simulink model "bidirection_buck_boost"  (R2025a)
settings: Solver=VariableStepAuto  StartTime=0.0  StopTime=0.05  MaxStep=1e-7  RelTol=1e-3
libraries: ee_lib x36, nesl_utility x29, fl_lib x26, spsPWMGeneratorDCDCLib x8, spsMeanLib x2, batteryecm_lib x1
settings Model: Creator=GNKRISHNAN  LastModifiedBy=GNKRISHNAN

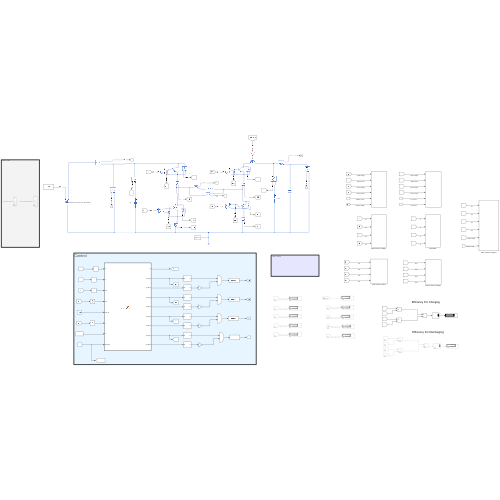
[thumbnail: Simulink's stored preview of the top-level diagram]
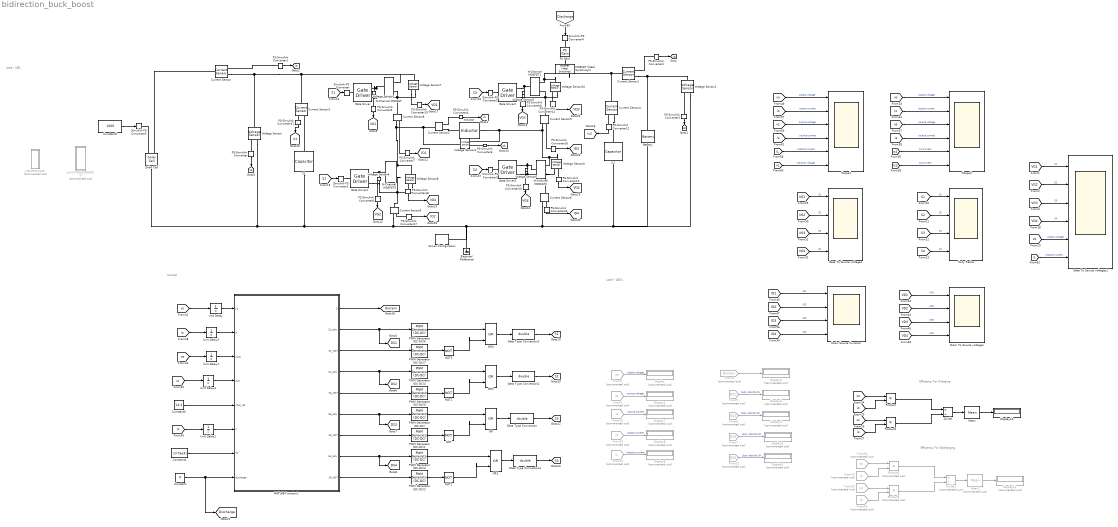
== system bidirection_buck_boost ==
  note: Load - LED
  note: Load - LED's
  note: Control
  note: Efficiency For Charging
  note: Efficiency For Discharging
  Battery : batteryecm_lib/Battery  Vnom=12 V  prm_dir=simscape.enum.battery.prm_dir.disabled  R1_dis=2 Ohm  R1_ch=2 Ohm  R1=4.9e-3 Ohm  prm_AH=simscape.enum.battery.prm_AH.infinite  AH=7.2 A*hr  V1=11.5 V  AH1=25 A*hr  prm_R2=simscape.enum.battery.prm_R2.disabled  R2=2000 Ohm  Tmeas=298.15 K  charge_measurement_port=simscape.enum.battery.enable.no  prm_dyn=simscape.enum.battery.prm_dyn.off  Rp1=0.005 Ohm  tau1=30 s  Rp2=0.005 Ohm  tau2=30 s  Rp3=0.005 Ohm  tau3=30 s  Rp4=0.005 Ohm  tau4=30 s  Rp5=0.005 Ohm  tau5=30 s  prm_fade=simscape.enum.battery.prm_fade.disabled  N_fade=100  AH_fade=45 A*hr  R1_fade=2.02 Ohm  R1_ch_fade=2.02 Ohm  V1_fade=10.35 V  prm_age=simscape.enum.battery.prm_age.disabled  prm_age_OCV=simscape.enum.battery.prm_age_OCV.OCV  OCV_age=0.9  SOC_age=60  Tmeas_age=298.15 K  delta_time_age_vec=[0] d  temperature_age_vec=[273] K  OCV_scaling_age=2.2134e6  OCV_offset_age=1.632e6  temp_exp_age=0.515833569 V  t_exp_age=0.75  Vnom_T2=12 V  R1_T2=2.2 Ohm  R1_T2_dis=2.2 Ohm  R1_T2_ch=2.2 Ohm  V1_T2=11.4 V  R2_T2=2200 Ohm  Rp1_T2=0.005 Ohm  tau1_T2=30 s  Rp2_T2=0.005 Ohm  tau2_T2=30 s  Rp3_T2=0.005 Ohm  tau3_T2=30 s  Rp4_T2=0.005 Ohm  tau4_T2=30 s  Rp5_T2=0.005 Ohm  tau5_T2=30 s  Tmeas2=273.15 K  thermal_port=simscape.enum.thermaleffects.omit  thermal_mass=30000 J/K  i_specify=off  i_priority=None  i=0 A  i_nominal_specify=off  i_nominal_value=1  i_nominal_unit=A  v_specify=off  v_priority=None  v=0 V  v_nominal_specify=off  v_nominal_value=1  v_nominal_unit=V  charge_specify=off  charge_priority=High  charge=50 A*hr  charge_nominal_specify=off  charge_nominal_value=1  charge_nominal_unit=A*hr  num_cycles_specify=off  num_cycles_priority=High  num_cycles=0  num_cycles_nominal_specify=off  num_cycles_nominal_value=1  num_cycles_nominal_unit=1  temperature_specify=off  temperature_priority=High  temperature=298.15 K  temperature_nominal_specify=off  temperature_nominal_value=1  temperature_nominal_unit=K
      settings: LibrarySourceBlock=batt_lib/Cells/Battery
  C1 : fl_lib/Electrical/Electrical Elements/Capacitor  c=100e-6 F  r=1e-6 Ohm  g=0 1/Ohm  i_specify=off  i_priority=High  i=1 A  i_nominal_specify=off  i_nominal_value=1  i_nominal_unit=A  v_specify=off  v_priority=Low  v=50 V  v_nominal_specify=off  v_nominal_value=1  v_nominal_unit=V  vc_specify=off  vc_priority=High  vc=50 V  vc_nominal_specify=off  vc_nominal_value=1  vc_nominal_unit=V
  C2 : fl_lib/Electrical/Electrical Elements/Capacitor  c=488e-6 F  r=1e-6 Ohm  g=0 1/Ohm  i_specify=off  i_priority=High  i=1 A  i_nominal_specify=off  i_nominal_value=1  i_nominal_unit=A  v_specify=off  v_priority=Low  v=12 V  v_nominal_specify=off  v_nominal_value=1  v_nominal_unit=V  vc_specify=off  vc_priority=High  vc=12 V  vc_nominal_specify=off  vc_nominal_value=1  vc_nominal_unit=V
  Constant : Constant  Value=0
  Constant4 : Constant  Value=1/(75e3)
  Constant5 : Constant  Value=1000
  Constant6 : Constant  Value=14.2
  Current Sensor{,1..6,8..9} (9 alike) : fl_lib/Electrical/Electrical Sensors/Current Sensor
  Data Type Conversion{,1..3} (4 alike) : DataTypeConversion  OutDataTypeStr=double  SaturateOnIntegerOverflow=off  RndMeth=Floor
  Display{,1..9,11} (11 alike) : Display  Commented=on
      Display11 settings: Format=bank
  Display10 : Display
      settings: Format=bank
  Divide : Product  Inputs=*/
  Divide1 : Product  Commented=on  Inputs=*/
  Drain Source Currents : Scope  NumInputPorts=4
      settings: ActiveDisplayString=4  ActiveDisplayYMinimum=-1.5306429258777277  ActiveDisplayYMaximum=0.21907576990254851  DataLoggingVariableName=ScopeData5
  Drain To Source voltages : Scope  NumInputPorts=4
      settings: ActiveDisplayYMinimum=-4.5564425884228816  ActiveDisplayYMaximum=38.582414890367822  DataLoggingVariableName=ScopeData4
  Duty Ratios : Scope  NumInputPorts=4
      settings: ActiveDisplayYMinimum=0.9  ActiveDisplayYMaximum=1.1
  Electrical Reference : fl_lib/Electrical/Electrical Elements/Electrical Reference
  From19 : From  Commented=on  GotoTag=is  TagVisibility=global
  From20 : From  Commented=on  GotoTag=io  TagVisibility=global
  From21 : From  Commented=on  GotoTag=iL  TagVisibility=global
  From22 : From  Commented=on  GotoTag=DS4  TagVisibility=global
  From4 : From  Commented=on  GotoTag=vo  TagVisibility=global
  From5 : From  Commented=on  GotoTag=vs  TagVisibility=global
  From51 : From  Commented=on  GotoTag=vs  TagVisibility=global
  From52 : From  Commented=on  GotoTag=is  TagVisibility=global
  From53 : From  Commented=on  GotoTag=vo  TagVisibility=global
  From54 : From  Commented=on  GotoTag=io  TagVisibility=global
  From6 : From  Commented=on  GotoTag=DS2  TagVisibility=global
  From7 : From  Commented=on  GotoTag=DS3  TagVisibility=global
  From8 : From  Commented=on  GotoTag=Dintern  TagVisibility=global
  From9 : From  Commented=on  GotoTag=DS1  TagVisibility=global
  Gate Driver{,1..3} (4 alike) : ee_lib/Semiconductors & Converters/Gate Driver  port_option=ee.enum.controlport.ps  uHigh=2.0 V  uLow=0.8 V  uHighValue=0.7  uLowValue=0.3  vHigh=15 V  vLow=0 V  tHigh=500 ns  tLow=0 ns  parameterization=ee.enum.semiconductors.gateDriverParam.outputImpedance  rHigh=2 Ohm  rLow=2 Ohm  tRise=20 ns  tFall=20 ns  cLoad=10 nF  ZonTime_specify=off  ZonTime_priority=None  ZonTime=0 s  ZoffTime_specify=off  ZoffTime_priority=None  ZoffTime=0 s
      settings: InternalSimscapePortConfiguration="{\"Bottom\":[],\"Left\":[{\"id\":\"u\",\"label\":\"u\",\"type\":\"input\"}],\"Right\":[{\"id\":\"G\",\"label\":\"G\",\"type\":\"foundation.electrical.electrical\"},{\"id\":\"S\",\"label\":\"S\",\"type\":\"foundation.electrical.electrical\"}],\"Top\":[]}"
  Gate To Source voltages : Scope  NumInputPorts=4
      settings: ActiveDisplayString=4  ActiveDisplayYMinimum=-2.1171010981224692  ActiveDisplayYMaximum=16.901953933343137  DataLoggingVariableName=ScopeData2
  Gate To Source voltages1 : Scope  NumInputPorts=6
      settings: ActiveDisplayString=6  ActiveDisplayYMinimum=-4.895588317884668  ActiveDisplayYMaximum=-0.48622530824491572
  Inductor : ee_lib/Passive/Inductor  l=150e-6 H  enable_L_tol=ee.enum.toleranceApplication.none  L_tol=20  tol_distribution=ee.enum.toleranceDistribution.uniform  nSigma=4  r=0 Ohm  g=1e-9 1/Ohm  enable_operating_limits=ee.enum.enable.no  operating_limit_action=ee.enum.passive.reportOpLim.warn  max_working_current=1 A  power_rating=1 W  i_L_specify=off  i_L_priority=High  i_L=2.5 A  i_L_nominal_specify=on  i_L_nominal_value=3  i_L_nominal_unit=A
  L1HZ-5780100000000 : Subsystem  Commented=on
  LXK2PW14V00 : Subsystem  Commented=on
      settings: PortSchema="{\"entries\":[{\"content\":{\"sides\":[{\"content\":{},\"type\":\"ConnectorPlacement.EquallySpacedRectSide\",\"uuid\":\"20fc5c96-5131-4911-af40-90c1653f2349\"},{\"content\":{\"side\":\"RIGHT\"},\"type\":\"ConnectorPlacement.EquallySpacedRectSide\",\"uuid\":\"84d94f68-b5bd-4d52-87d0-e2c404d7394b\"},{\"content\":{\"connectorIds\":[\"LConn1\"],\"side\":\"TOP\"},\"type\":\"ConnectorPlacement.EquallySpacedRectSide\",\"uuid\":\"fbb55fab-e1b4-4776-8e6f-d36497a875a9\"},{\"content\":{\"connectorIds\":[\"RConn1\"],\"side\":\"BOTTOM\"},\"type\":\"ConnectorPlacement.EquallySpacedRectSide\",\"uuid\":\"0f47366a-6e94-42f9-9b64-329c1064e3d3\"}]},\"type\":\"ConnectorPlacement.EquallySpacedConnector\",\"uuid\":\"9fc36618-202f-478c-8e37-58b0074959b4\"}],\"packageUris\":[\"http://schema.mathworks.com/mf0/Connector/R2020b\"],\"version\":\"1.0\"}"
  MATLAB Function1 : MATLAB Function  TreatAsAtomicUnit=on  SystemSampleTime=1/(75e3)
  "MOSFET (Ideal, Switching)4" : ee_lib/Semiconductors & Converters/MOSFET (Ideal, Switching)  port_option=ee.enum.controlport.ps  Rds=0.01 Ohm  Goff=1e-6 1/Ohm  Vth=0.5 V  diode_param=ee.enum.semiconductors.protectionDiode.nodynamics  diode_Vf=0.8 V  diode_Ron=0.001 Ohm  diode_Goff=1e-5 1/Ohm  diode_C=50e-9 F  diode_iRM=-235 A  diode_iF=300 A  diode_idot=-50 A/us  diode_trr_param=ee.enum.converters.diodeReverseParam.trr_factor  diode_trr_factor=3  diode_trr=15 us  diode_Qrr=1500 s*uA  ids_specify=off  ids_priority=None  ids=0 A  ids_nominal_specify=off  ids_nominal_value=1  ids_nominal_unit=A  vds_specify=off  vds_priority=None  vds=0 V  vds_nominal_specify=off  vds_nominal_value=1  vds_nominal_unit=V  vgs_specify=off  vgs_priority=None  vgs=0 V  vgs_nominal_specify=off  vgs_nominal_value=1  vgs_nominal_unit=V  thermal_loss_option=ee.enum.converters.thermalLossOption.constantvalues  Von_data=[0, 1.8, 3.2, 6, 10, 16; 0, 2, 5.5, 9.5, 15, 25] V  Tj=[298.15, 448.15] K  Iout_data=[0, 20, 40, 60, 80, 100] A  Eon_data=[0, 55.04, 124.57, 235.53, 362.12; 0, 71.25, 161.25, 304.88, 468.75] * 1e-6 J  Eoff_data=[0, 18, 30, 56.1, 76.5; 0, 22.5, 37.5, 70.13, 95.63] * 1e-6 J  Eon_data_3D=[zeros(2, 5, 3)] J  Eoff_data_3D=[zeros(2, 5, 3)] J  Tj_loss=[298.15, 448.15] K  Iout_data_loss=[0, 10, 20, 30, 40] A  tabulateWithVds=false  Vds_loss=[0, 150, 300] V  Eon_scalar=22.86e-3 J  Eoff_scalar=17.14e-3 J  Voff=300 V  Iout_scalar=600 A  useCurrentFromPreviousCycle=false  useVoltageFromPreviousCycle=false  diodeModelType=ee.enum.converters.diodeModelType.pwl  diodeTableType=ee.enum.diode.tableType.IfMat  diode_ReverseIVType=ee.enum.diode.diodeReverseIV.constant  diode_IfMat=[.07, .12, .19, 1.75, 4.24, 7.32, 11.2; .16, .3, .72, 2.14, 4.02, 6.35, 9.12] A  diode_VfMat=[.9, 1.15, 1.25, 1.5, 1.75, 2.17, 2.6, 2.85; .58, .68, .75, 1.1, 1.38, 1.77, 2.27, 2.7] V  diode_TjVec=[25, 125] degC  diode_VfVec=[.5, .7, .9, 1.3, 1.7, 2.1, 2.5] V  diode_IfVec=[.1, .2, .5, 1, 2, 4, 7, 10] A  diode_IrMat=[1e-06, 2e-06, 5e-06, 1e-05, 2.5e-05, 5e-05, .0001; 2e-06, 5e-06, 1e-05, 4e-05, 8e-05, .0002, .0005] A  diode_VrMat=[10, 100, 200, 250, 300, 325, 350; 10, 70, 160, 220, 270, 300, 320] V  diode_VrVec=[10, 20, 40, 50, 70, 80, 100] V  diode_IrVec=[1e-06, 2e-06, 5e-06, 1e-05, 2e-05, 5e-05, .0001] A  diode_Vr=-600 V  diode_Ls=150 nH  diode_Erec=0.03 J  diode_rec_loss_model=ee.enum.diode.reverseRecoveryModel.fixed  diode_ErecVal=0 J  diode_scaleWithIandV=true  diode_ErecMat=zeros(2, 3) J  diode_TjrecVec=[298.15, 398.15] K  diode_IfrecVec=[.1, 1, 10] A  diode_IrecVal=10 A  diode_VrecVal=10 V  diode_tFilter=1 / 1000 / 100 s  separateThermalPortForDiode=false  thermal_network_parameterization=ee.enum.thermalNetworkTopology.external  Rth=[.03, .2] K/W  Rth_Cauer=[.03, .1, .2] K/W  Rth_Foster=[.08, .14, .22, .16] K/W  thermal_mass_parameterization=ee.enum.thermalNetwork.timeconstant  thermal_mass=[3, 25] J/K  thermal_mass_Cauer=[3, 10, 25] J/K  thermal_mass_Foster=[.001, .005, .05, .5] J/K  thermal_time_constant=[.1, 5] s  thermal_time_constant_Cauer=[.1, 1, 5] s  thermal_time_constant_Foster=[7e-05, .0007, .01, .08] s  thermal_mass_initial_temperatures=[25, 25] degC  thermal_mass_initial_temperatures_Cauer=[25, 25, 25] degC  junction_thermal_mass=0.1 J/K  Tvec_initial_Foster=[25, 25, 25, 25] degC  RthDiode=[.03, .2] K/W  RthCauerDiode=[.03, .1, .2] K/W  RthFosterDiode=[.03, .2] K/W  thermalMassDiode=[3, 25] J/K  thermalMassCauerDiode=[3, 10, 25] J/K  thermalMassFosterDiode=[33, 50] J/K  thermalTauDiode=[.1, 5] s  thermalTauCauerDiode=[.1, 1, 5] s  thermalTauFosterDiode=[1, 10] s  thermalMassInitTempDiode=[25, 25] degC  thermalMassInitTempCauerDiode=[25, 25, 25] degC  junctionthermalMassDiode=0.1 J/K  TVecInitialFosterDiode=[25, 25, 25, 25] degC  no_thermal_network=0  mosfet_junction_temperature_specify=off  mosfet_junction_temperature_priority=None  mosfet_junction_temperature=25 degC  mosfet_junction_temperature_nominal_specify=off  mosfet_junction_temperature_nominal_value=1  mosfet_junction_temperature_nominal_unit=degC  diode_junction_temperature_specify=off  diode_junction_temperature_priority=None  diode_junction_temperature=25 degC  diode_junction_temperature_nominal_specify=off  diode_junction_temperature_nominal_value=1  diode_junction_temperature_nominal_unit=degC  Qj_specify=off  Qj_priority=None  Qj=0 W  Qj_nominal_specify=off  Qj_nominal_value=1  Qj_nominal_unit=W  accumulatedSwitchingLosses_specify=off  accumulatedSwitchingLosses_priority=None  accumulatedSwitchingLosses=0 J
  Mean : spsMeanLib/Mean  Freq=100e3  Vinit=0.5  Ts=0
  Mean1 : spsMeanLib/Mean  Commented=on  Freq=100e3  Vinit=0.5  Ts=0
  N-Channel MOSFET{,1..3} (4 alike) : ee_lib/Semiconductors & Converters/N-Channel MOSFET  paramTerminal=ee.enum.mosfet.numberOfTerminals.three  parameterization=ee.enum.mosfet.parameterization.datasheet  Beta=5.0 A/V^2  Rds=17.5 mOhm  Id=49.0 A  Vgs=20 V  Vth=4.0 V  Vth0=1.7 V  lam=0 1/V  gamma_vth=0.5 V^(1/2)  phib=0.5 V  Vth1=1.9071 V  Vbs1=-1 V  Vth2=2.066 V  Vbs2=-2 V  Tmeas=25 degC  Vgs_vec=[-1, -.5, 2, 3, 4, 5] V  Vds_vec=[0, 2, 4, 8, 12, 16, 20] V  Vbs_vec=[0, -4, -6, -12] V  T_vec=[25, 125] degC  Vth_vec=[.4, 1.2, 1.4, 1.45] V  Vth_mat=[.4, .35; 1.2, 1.15; 1.4, 1.35; 1.45, 1.4] V  Ids_mat=[0, 0, 0, 0, 0, 0, 0; 0, 0, 0, 0, 0, 0, 0; 0, .003, .0038, .0043, .0046, .0048, .0049; 0, .0055, .008, .009, .0095, .01, .0101; 0, .0115, .016, .018, .019, .0195, .02; 0, .0152, .0225, .0265, .028, .0295, .03] A  Ids_mat0=[0, 0, 0, 0, 0, 0, 0; 0, 0, 0, 0, 0, 0, 0; 0, .003, .0038, .0043, .0046, .0048, .0049; 0, .0055, .008, .009, .0095, .01, .0101; 0, .0115, .016, .018, .019, .0195, .02; 0, .0152, .0225, .0265, .028, .0295, .03] A  Ids_mat_3D=zeros(6, 7, 2) A  Ids_mat_3D0=zeros(6, 7, 2) A  IV_table_symmetry=ee.enum.mosfet.symmetricNIV.no  RS=0.0001 Ohm  RD=0.01 Ohm  RB=0.001 Ohm  LeadRs=0 Ohm  LeadRd=0 Ohm  LeadRg=0 Ohm  LeadRb=0 Ohm  LS=0 nH  LD=0 nH  LG=0 nH  LB=0 nH  C_param=ee.enum.mosfet.capacitanceParam.fixedciss  C_GS=270 pF  C_GD=80 pF  C_GB=0 pF  C_DS=0 pF  C_iss=1470 pF  C_rss=88 pF  C_oss=360 pF  C_iss_vec=[720, 700, 590, 470, 390, 310] pF  C_rss_vec=[450, 400, 300, 190, 95, 55] pF  C_oss_vec=[900, 810, 690, 420, 270, 170] pF  C_GS_vec=[270, 300, 290, 280, 295, 255] pF  C_GD_vec=[450, 400, 300, 190, 95, 55] pF  C_GB_vec=[270, 300, 290, 280, 295, 255] pF  C_Vgs_vec=0 V  C_DS_vec=[450, 410, 390, 230, 175, 115] pF  C_Vds_vec=[.1, .3, 1, 3, 10, 30] V  V_GS_for_cap_data=0 V  charge_linearity_param=ee.enum.mosfet.cgdLinearity.constant  C_OX=200 pF  V_C_OX=-0.5 V  charge_linearity_param_vgb=ee.enum.mosfet.cgbLinearity.instantly  charge_linearity_param_with_vgb=ee.enum.mosfet.cgbLinearityWithSeparateCgb.instantly  Di_param=ee.enum.mosfet.diodeParam.no  IsDiode=1e-12 A  Vbi=0.6 V  n=1  Cj0Diode=0 pF  TT=50e-9 s  Tmeas_dio=25 degC  TableTypeNoT=ee.enum.mosfet.tableType.IfMat  TableType=ee.enum.diode.tableType.IfMat  IfVec=[.07, .12, .19, 1.75, 4.24, 7.32, 11.2] A  IfMat=[.07, .12, .19, 1.75, 4.24, 7.32, 11.2; .16, .3, .72, 2.14, 4.02, 6.35, 9.12] A  VfVecV=[.9, 1.15, 1.25, 1.5, 1.75, 2.17, 2.6, 2.85] V  VfMatV=[.9, 1.15, 1.25, 1.5, 1.75, 2.17, 2.6, 2.85; .58, .68, .75, 1.1, 1.38, 1.77, 2.27, 2.7] V  TjVec=[25, 125] degC  VfVec=[.5, .7, .9, 1.3, 1.7, 2.1, 2.5] V  IfVecV=[.1, .2, .5, 1, 2, 4, 7, 10] A  diode_Goff=1e-12 1/Ohm  prmDatasheet=ee.enum.temperatureParameterization.none  prmEquCoeff=ee.enum.temperatureParameterization.none  dVth_dT=-6 mV/K  dVth0_dT=-6 mV/K  Rds_T2=0.037 Ohm  BEXDatasheet=-1.5  BEXEquCoeff=-1.5  etaisDatasheet=3  etaisEquCoeff=3  Tmeas2=125 degC  etaisTabulated=3  TdeviceDatasheet=25 degC  TdeviceEquCoeff=25 degC  TdeviceTabulated=25 degC  i_g_specify=off  i_g_priority=None  i_g=0 A  i_g_nominal_specify=off  i_g_nominal_value=1  i_g_nominal_unit=A  i_d_specify=off  i_d_priority=None  i_d=0 A  i_d_nominal_specify=off  i_d_nominal_value=1  i_d_nominal_unit=A  i_b_specify=off  i_b_priority=None  i_b=0 A  i_b_nominal_specify=off  i_b_nominal_value=1  i_b_nominal_unit=A  voltage_gs_specify=off  voltage_gs_priority=None  voltage_gs=0 V  voltage_gs_nominal_specify=off  voltage_gs_nominal_value=1  voltage_gs_nominal_unit=V  voltage_ds_specify=off  voltage_ds_priority=None  voltage_ds=0 V  voltage_ds_nominal_specify=off  voltage_ds_nominal_value=1  voltage_ds_nominal_unit=V  voltage_bs_specify=off  voltage_bs_priority=None  voltage_bs=0 V  voltage_bs_nominal_specify=off  voltage_bs_nominal_value=1  voltage_bs_nominal_unit=V  v_Cgs_specify=off  v_Cgs_priority=High  v_Cgs=0 V  v_Cgs_nominal_specify=off  v_Cgs_nominal_value=1  v_Cgs_nominal_unit=V  v_Cds_specify=off  v_Cds_priority=High  v_Cds=0 V  v_Cds_nominal_specify=off  v_Cds_nominal_value=1  v_Cds_nominal_unit=V  v_Cbs_specify=off  v_Cbs_priority=High  v_Cbs=0 V  v_Cbs_nominal_specify=off  v_Cbs_nominal_value=1  v_Cbs_nominal_unit=V  thermal_network_parameterization=ee.enum.thermalNetworkTopology.junctionCase  Rth=[0, 10] K/W  Rth_Cauer=[1, 3, 10] K/W  Rth_Foster=[.08, .14, .22, .16] K/W  thermal_mass_parameterization=ee.enum.thermalNetwork.timeconstant  thermal_mass=[0, 1] J/K  thermal_mass_Cauer=[.1, .3, 1] J/K  thermal_mass_Foster=[.001, .005, .05, .5] J/K  thermal_time_constant=[0, 10] s  thermal_time_constant_Cauer=[1, 3, 10] s  thermal_time_constant_Foster=[7e-05, .0007, .01, .08] s  thermal_mass_initial_temperatures=[25, 25] degC  thermal_mass_initial_temperatures_Cauer=[25, 25, 25] degC  Tvec_initial_Foster=[25, 25, 25, 25] degC  betaref=18 A/V^2  Vfbref=-1.1 V  gamma=3.5 V^(1/2)  phib2ref=1 V  thesatref=0.4 1/V  alpha=0  Vp=5e-2 V  thesrref=0 1/V  m=8  Tref=25 degC  Rsref=2e-3 Ohm  Rdref=0.17 Ohm  Rgref=8.4 Ohm  Rbref=2e-3 Ohm  Cox=1500 pF  Cgso=100 pF  Cgdo=14 pF  Isref=5.2e-13 A  Cj0=480 pF  Tprm=1  etabet=1.3  Stvfb=5e-4 V/K  Stphib=-8.5e-4 V/K  etasat=1.04  etasr=0.65  etar=0.95  etais=3  Tsim=25 degC  Ig_specify=off  Ig_priority=None  Ig=0 A  Ig_nominal_specify=off  Ig_nominal_value=1  Ig_nominal_unit=nA  Ids_specify=off  Ids_priority=None  Ids=0 A  Ids_nominal_specify=off  Ids_nominal_value=1  Ids_nominal_unit=A  Ib_specify=off  Ib_priority=None  Ib=0 A  Ib_nominal_specify=off  Ib_nominal_value=1  Ib_nominal_unit=uA  V_gs_specify=off  V_gs_priority=None  V_gs=0 V  V_gs_nominal_specify=off  V_gs_nominal_value=1  V_gs_nominal_unit=V  V_ds_specify=off  V_ds_priority=None  V_ds=0 V  V_ds_nominal_specify=off  V_ds_nominal_value=1  V_ds_nominal_unit=V  V_bs_specify=off  V_bs_priority=None  V_bs=0 V  V_bs_nominal_specify=off  V_bs_nominal_value=1  V_bs_nominal_unit=V  QGoverCox_specify=off  QGoverCox_priority=None  QGoverCox=0 V  QGoverCox_nominal_specify=off  QGoverCox_nominal_value=1  QGoverCox_nominal_unit=V  QDoverCox_specify=off  QDoverCox_priority=None  QDoverCox=0 V  QDoverCox_nominal_specify=off  QDoverCox_nominal_value=1  QDoverCox_nominal_unit=V  QBoverCox_specify=off  QBoverCox_priority=None  QBoverCox=0 V  QBoverCox_nominal_specify=off  QBoverCox_nominal_value=1  QBoverCox_nominal_unit=V  T0=[25, 25] degC  T0_Cauer=[25, 25, 25] degC
  NOT{,1..3} (4 alike) : Logic  Operator=NOT  IconShape=distinctive  AllPortsSameDT=off  OutDataTypeStr=boolean
  OR{,1..3} (4 alike) : Logic  Operator=OR  IconShape=distinctive  AllPortsSameDT=off  OutDataTypeStr=boolean
  PS Gain : fl_lib/Physical Signals/Functions/PS Gain  gain=10 V
  PS-Simulink Converter{,1..12,14..20} (20 alike) : nesl_utility/PS-Simulink Converter  PhysicalDomain=network_engine_domain  SubClassName=ps_output  LeftPortType=input  RightPortType=output  PseudoPeriodic=off  Frequencies=[]  VectorFormat=inherit  Unit=inherit  AffineConversion=off
  PWM Generator (DC-DC){,1..7} (8 alike) : spsPWMGeneratorDCDCLib/PWM Generator (DC-DC)  Fsw=75e3  Ts=0
  Product : Product
  Product1 : Product
  Product2 : Product  Commented=on
  Product3 : Product  Commented=on
  Scope1 : Scope  NumInputPorts=6
      settings: ActiveDisplayString=5  ActiveDisplayYMinimum=-17.405950682168605  ActiveDisplayYMaximum=156.65355621450624  DataLoggingVariableName=ScopeData6
  Scope3 : Scope  NumInputPorts=6
      settings: ActiveDisplayYMinimum=-1.5694108173115382  ActiveDisplayYMaximum=14.126143121517581  DataLoggingVariableName=ScopeData3
  Simulink-PS Converter{,1..5} (6 alike) : nesl_utility/Simulink-PS Converter  PhysicalDomain=network_engine_domain  SubClassName=ps_input  LeftPortType=input  RightPortType=output  PseudoPeriodic=off  Frequencies=[]  NoiseDistribution=none  NoiseParameters=[]  Unit=1  AffineConversion=off  FilteringAndDerivatives=provide  SimscapeFilterOrder=1  InputFilterTimeConstant=0.001  UdotUserProvided=0
  Solar Cell : ee_lib/Sources/Solar Cell  PartSpecification="{\"CollectionId\":\"SimscapeElectrical\",\"CollectionVersion\":\"1.0.0\",\"DatasetId\":\"Mitsubishi_Electric|PV_MLU250HC|simscape.electrical.solarCell\",\"DisplayName\":\"Mitsubishi_Electric:PV_MLU250HC\"}"  prm=3  Isc=4.395 % Datasheet derived A  Voc=0.62698 % Datasheet derived V  Is=3.90785352555275e-07 % Datasheet derived A  Is2=2.03851654351426e-09 % Datasheet derived A  Iph=4.39501564800196 % Datasheet derived A  Ir0=1000 % Datasheet derived W/m^2  ec=1.50308795420873 % Datasheet derived  N2=1.46170678478288 % Datasheet derived  Rs=0.00316744030774209 % Datasheet derived Ohm  Rp=887.270164200596 % Datasheet derived Ohm  N_series=60 % Datasheet derived  N_parallel=2 % Datasheet derived  TIPH1=0.000560046095116037 % Datasheet derived 1/K  EG=1.12 % Datasheet derived eV  TXIS1=6.0075926142096 % Datasheet derived  TXIS2=15.9012627985887 % Datasheet derived  TRS1=0.216297310987677 % Datasheet derived  TRP1=0 % Parameter not set  Tmeas=25 % Datasheet derived degC  TFIXED=25 % Datasheet derived degC  thermal_mass=100 % Parameter not set J/K  initial_temperature=25 degC
      settings: AttributesFormatString=Mitsubishi_Electric:PV_MLU250HC
  Solver Configuration : nesl_utility/Solver Configuration  PhysicalDomain=network_engine_domain  SubClassName=solver  LeftPortType=input  RightPortType=generic  Tones=[]  Harmonics=[]  SimulateNoise=off  Profile=off  UseLocalSampling=off  EnableSwitchedLinearOptims=on  FrequencyDomain=off  UseCCode=off  RelTol=0.001  AbsTol=0.001  MinStep=1e-09  ToWorkspace=off  RevertToSquareIcSolve=off  NumHomotopyIterations=100  PhasorMode=off  PhasorModeNumHarmonics=1  ConsistencySolver=NEWTON_XTOL_AFTER_FTOL  IndexReductionMethod=DerivativeReplacement  DoDC=off  ResidualTolerance=1e-09  ConsistencyTolSource=GLOBAL  ConsistencyAbsTol=0.001  ConsistencyRelTol=0.001  ConsistencyTolFactor=0.001  UseLocalSolver=off  LocalSolverChoice=NE_BACKWARD_EULER_ADVANCER  ResolveIndetEquations=on  FunctionEvalNumThread=1  LocalSolverSampleTime=0.001  DoFixedCost=off  MaxNonlinIter=3  MaxModeIter=2  ComputeImpulses=off  ImpulseIterations=2  LinearAlgebra=auto  LinearAlgebraNumThread=0  EquationFormulation=NE_TIME_EF  DelaysMemoryBudget=1024  AutomaticFiltering=on  FilteringTimeConstant=0.001  PartitionStorageMethod=AS_NEEDED  PartitionMemoryBudget=1024  PartitionMethod=ROBUST  MultibodyUseLocalSolver=off  MultibodyLocalSolverChoice=ODE1  MultibodyLocalSolverSampleTime=0.001
  Unit Delay{,1..4} (5 alike) : UnitDelay  SampleTime=-1  HasFrameUpgradeWarning=on
  Voltage Sensor{,1..10} (11 alike) : fl_lib/Electrical/Electrical Sensors/Voltage Sensor
  tag scope: DS1=global, DS2=global, DS3=global, DS4=global, Dintern=global, Discharge=global, ID1=global, ID2=global, ID3=global, ID4=global, S1=global, S2=global, S3=global, S4=global, VD1=global, VD2=global, VD3=global, VD4=global, VG1=global, VG2=global, VG3=global, VG4=global, iL=global, ic1=global, ic2=global, io=global, is=global, vL=global, vo=global, vs=global
  wires:
  From6/1 -> Display4/1  "Duty ratio for S2"
  From22/1 -> Display6/1  "Duty ratio for S4"
  [S2] -> Duty Ratios/2  "S2"
  Unit Delay/1 -> MATLAB Function1/1(Vs)
  From8/1 -> Display2/1
  MATLAB Function1/8(S4_duty) -> PWM Generator (DC-DC)3/1, [DS4]
  Unit Delay1/1 -> MATLAB Function1/3(Vout)
  [vo] -> Unit Delay1/1
  [S1] -> Simulink-PS Converter/1
  [S4] -> Duty Ratios/4  "S4"
  [S3] -> Simulink-PS Converter2/1
  Constant4/1 -> MATLAB Function1/7(Ts)
  PS-Simulink Converter2/1 -> [vo]
  PS-Simulink Converter1/1 -> [is]
  [vs] -> Unit Delay/1
  [S1] -> Duty Ratios/1  "S1"
  Unit Delay2/1 -> MATLAB Function1/6(Il)
  PS-Simulink Converter4/1 -> [iL]
  [S3] -> Duty Ratios/3  "S3"
  From9/1 -> Display3/1  "Duty ratio for S1"
  [iL] -> Unit Delay2/1
  From4/1 -> Display/1  "output voltage"
  MATLAB Function1/6(S3_duty) -> PWM Generator (DC-DC)/1, [DS3]
  [S4] -> Simulink-PS Converter3/1
  PS-Simulink Converter/1 -> [vs]
  PS-Simulink Converter3/1 -> [io]
  From7/1 -> Display5/1  "Duty ratio for S3"
  From5/1 -> Display1/1  "source voltage"
  [S2] -> Simulink-PS Converter1/1
  From20/1 -> Display8/1  "output current"
  From19/1 -> Display7/1  "source current"
  From21/1 -> Display9/1  "inductor current"
  PS-Simulink Converter5/1 -> [VG1]
  PS-Simulink Converter6/1 -> [vL]
  Constant5/1 -> Simulink-PS Converter5/1
  [vo] -> Product/1
  [io] -> Product/2
  [is] -> Product1/2
  [vs] -> Product1/1
  Divide/1 -> Mean/1
  Constant6/1 -> MATLAB Function1/5(Vout_ref)
  Mean/1 -> Display10/1
  PS-Simulink Converter8/1 -> [VG2]
  PS-Simulink Converter9/1 -> [VG3]
  PS-Simulink Converter10/1 -> [VG4]
  [VG3] -> Gate To Source voltages/3  "S3"
  [VG1] -> Gate To Source voltages/1  "S1"
  [VG4] -> Gate To Source voltages/4  "S4"
  [VG2] -> Gate To Source voltages/2  "S2"
  PS-Simulink Converter11/1 -> [ic1]
  PS-Simulink Converter12/1 -> [ic2]
  PS-Simulink Converter19/1 -> [VD1]
  PS-Simulink Converter18/1 -> [VD2]
  PS-Simulink Converter14/1 -> [VD3]
  PS-Simulink Converter15/1 -> [VD4]
  PS-Simulink Converter16/1 -> [ID3]
  PS-Simulink Converter17/1 -> [ID2]
  [VD4] -> Drain To Source voltages/4  "VD4"
  [VD3] -> Drain To Source voltages/3  "VD3"
  [VD2] -> Drain To Source voltages/2  "VD2"
  [VD1] -> Drain To Source voltages/1  "VD1"
  [ID1] -> Drain Source Currents/1  "ID1"
  [ID2] -> Drain Source Currents/2  "ID2"
  [ID3] -> Drain Source Currents/3  "ID3"
  [ID4] -> Drain Source Currents/4  "ID4"
  Constant/1 -> [Discharge], MATLAB Function1/8(discharge)
  MATLAB Function1/1(D) -> [Dintern]
  [is] -> Unit Delay3/1
  Unit Delay3/1 -> MATLAB Function1/2(Is)
  [io] -> Unit Delay4/1
  Unit Delay4/1 -> MATLAB Function1/4(Iout)
  Product/1 -> Divide/1
  Product1/1 -> Divide/2
  MATLAB Function1/4(S2_duty) -> PWM Generator (DC-DC)4/1, [DS2]
  MATLAB Function1/2(S1_duty) -> PWM Generator (DC-DC)6/1, [DS1]
  MATLAB Function1/7(S3_NOT) -> PWM Generator (DC-DC)1/1
  PWM Generator (DC-DC)1/1 -> NOT/1
  NOT/1 -> OR/2
  PWM Generator (DC-DC)/1 -> OR/1
  OR/1 -> Data Type Conversion/1
  Data Type Conversion/1 -> [S3]
  NOT1/1 -> OR1/2
  PWM Generator (DC-DC)2/1 -> NOT1/1
  MATLAB Function1/9(S4_NOT) -> PWM Generator (DC-DC)2/1
  Data Type Conversion1/1 -> [S4]
  OR1/1 -> Data Type Conversion1/1
  PWM Generator (DC-DC)3/1 -> OR1/1
  PWM Generator (DC-DC)4/1 -> OR2/1
  MATLAB Function1/5(S2_NOT) -> PWM Generator (DC-DC)5/1
  PWM Generator (DC-DC)5/1 -> NOT2/1
  NOT2/1 -> OR2/2
  OR2/1 -> Data Type Conversion2/1
  Data Type Conversion2/1 -> [S2]
  PWM Generator (DC-DC)6/1 -> OR3/1
  MATLAB Function1/3(S1_NOT) -> PWM Generator (DC-DC)7/1
  PWM Generator (DC-DC)7/1 -> NOT3/1
  NOT3/1 -> OR3/2
  OR3/1 -> Data Type Conversion3/1
  Data Type Conversion3/1 -> [S1]
  Product3/1 -> Divide1/2
  Product2/1 -> Divide1/1
  Mean1/1 -> Display11/1
  Divide1/1 -> Mean1/1
  From53/1 -> Product3/1
  From54/1 -> Product3/2
  From52/1 -> Product2/2
  From51/1 -> Product2/1
  [Discharge] -> Simulink-PS Converter4/1
  PS-Simulink Converter7/1 -> [ID1]
  PS-Simulink Converter20/1 -> [ID4]
  [vL] -> Scope1/6  "inductor voltage"
  [io] -> Scope1/2  "output current"
  [iL] -> Scope1/5  "inductor curent"
  [vo] -> Scope1/1  "output voltage"
  [is] -> Scope1/4  "source current"
  [vs] -> Scope1/3  "source voltage"
  [io] -> Scope3/2  "output current"
  [ic2] -> Scope3/6  "C2 Current"
  [is] -> Scope3/4  "source current"
  [vs] -> Scope3/3  "source voltage"
  [vo] -> Scope3/1  "output voltage"
  [ic1] -> Scope3/5  "C1 Current"
  [VG2] -> Gate To Source voltages1/2  "S2"
  [VG4] -> Gate To Source voltages1/4  "S4"
  [VG1] -> Gate To Source voltages1/1  "S1"
  [VG3] -> Gate To Source voltages1/3  "S3"
  [vo] -> Gate To Source voltages1/5  "output voltage"
  [iL] -> Gate To Source voltages1/6  "inductor curent"
  connections:
  Voltage Sensor/LConn1 -- Current Sensor/RConn2 -- Voltage Sensor7/LConn1 -- N-Channel MOSFET/RConn1 -- Current Sensor3/LConn1
  Current Sensor1/RConn2 -- Battery/LConn1 -- Voltage Sensor1/LConn1
  Current Sensor9/LConn1 -- Voltage Sensor10/RConn2 -- Voltage Sensor5/RConn2 -- Gate Driver2/RConn2 -- N-Channel MOSFET1/RConn2
  PS-Simulink Converter4/LConn1 -- Current Sensor2/RConn1
  N-Channel MOSFET3/LConn1 -- Voltage Sensor4/LConn1 -- Gate Driver1/RConn1
  Gate Driver2/RConn1 -- Voltage Sensor5/LConn1 -- N-Channel MOSFET1/LConn1
  Current Sensor2/RConn2 -- Inductor/LConn1
  Gate Driver3/RConn1 -- Voltage Sensor6/LConn1 -- N-Channel MOSFET2/LConn1
  PS-Simulink Converter3/LConn1 -- Current Sensor1/RConn1
  Simulink-PS Converter1/RConn1 -- Gate Driver1/LConn1
  Gate Driver3/LConn1 -- Simulink-PS Converter3/RConn1
  PS-Simulink Converter1/LConn1 -- Current Sensor/RConn1
  Gate Driver/LConn1 -- Simulink-PS Converter/RConn1
  Simulink-PS Converter2/RConn1 -- Gate Driver2/LConn1
  PS-Simulink Converter2/LConn1 -- Voltage Sensor1/RConn1
  Voltage Sensor2/LConn1 -- N-Channel MOSFET/LConn1 -- Gate Driver/RConn1
  PS-Simulink Converter/LConn1 -- Voltage Sensor/RConn1
  Voltage Sensor2/RConn1 -- PS-Simulink Converter5/LConn1
  PS-Simulink Converter6/LConn1 -- Voltage Sensor3/RConn1
  Solar Cell/LConn1 -- Simulink-PS Converter5/RConn1
  Current Sensor1/LConn1 -- "MOSFET (Ideal, Switching)4"/RConn1 -- Current Sensor4/LConn1
  Voltage Sensor/RConn2 -- Solar Cell/RConn1 -- C1/RConn1 -- Current Sensor5/RConn2 -- Electrical Reference/LConn1 -- Solver Configuration/RConn1 -- Voltage Sensor1/RConn2 -- Battery/RConn1 -- C2/RConn1 -- Current Sensor6/RConn2
  Voltage Sensor10/LConn1 -- N-Channel MOSFET1/RConn1 -- "MOSFET (Ideal, Switching)4"/RConn2
  Voltage Sensor4/RConn1 -- PS-Simulink Converter8/LConn1
  PS-Simulink Converter9/LConn1 -- Voltage Sensor5/RConn1
  PS-Simulink Converter10/LConn1 -- Voltage Sensor6/RConn1
  C1/LConn1 -- Current Sensor3/RConn2
  PS-Simulink Converter11/LConn1 -- Current Sensor3/RConn1
  Current Sensor4/RConn2 -- C2/LConn1
  PS-Simulink Converter12/LConn1 -- Current Sensor4/RConn1
  Current Sensor2/LConn1 -- N-Channel MOSFET3/RConn1 -- Voltage Sensor8/LConn1 -- Current Sensor8/RConn2 -- Voltage Sensor3/LConn1
  Inductor/RConn1 -- Voltage Sensor9/LConn1 -- N-Channel MOSFET2/RConn1 -- Current Sensor9/RConn2 -- Voltage Sensor3/RConn2
  PS-Simulink Converter14/LConn1 -- Voltage Sensor10/RConn1
  PS-Simulink Converter15/LConn1 -- Voltage Sensor9/RConn1
  PS-Simulink Converter16/LConn1 -- Current Sensor9/RConn1
  PS-Simulink Converter18/LConn1 -- Voltage Sensor8/RConn1
  Voltage Sensor7/RConn1 -- PS-Simulink Converter19/LConn1
  PS Gain/LConn1 -- Simulink-PS Converter4/RConn1
  PS Gain/RConn1 -- "MOSFET (Ideal, Switching)4"/LConn1
  Voltage Sensor8/RConn2 -- Gate Driver1/RConn2 -- Voltage Sensor4/RConn2 -- Current Sensor5/LConn1 -- N-Channel MOSFET3/RConn2
  PS-Simulink Converter17/LConn1 -- Current Sensor5/RConn1
  PS-Simulink Converter7/LConn1 -- Current Sensor8/RConn1
  Gate Driver3/RConn2 -- Voltage Sensor9/RConn2 -- N-Channel MOSFET2/RConn2 -- Current Sensor6/LConn1 -- Voltage Sensor6/RConn2
  PS-Simulink Converter20/LConn1 -- Current Sensor6/RConn1
  Voltage Sensor2/RConn2 -- N-Channel MOSFET/RConn2 -- Current Sensor8/LConn1 -- Voltage Sensor7/RConn2 -- Gate Driver/RConn2
  Solar Cell/LConn2 -- Current Sensor/LConn1

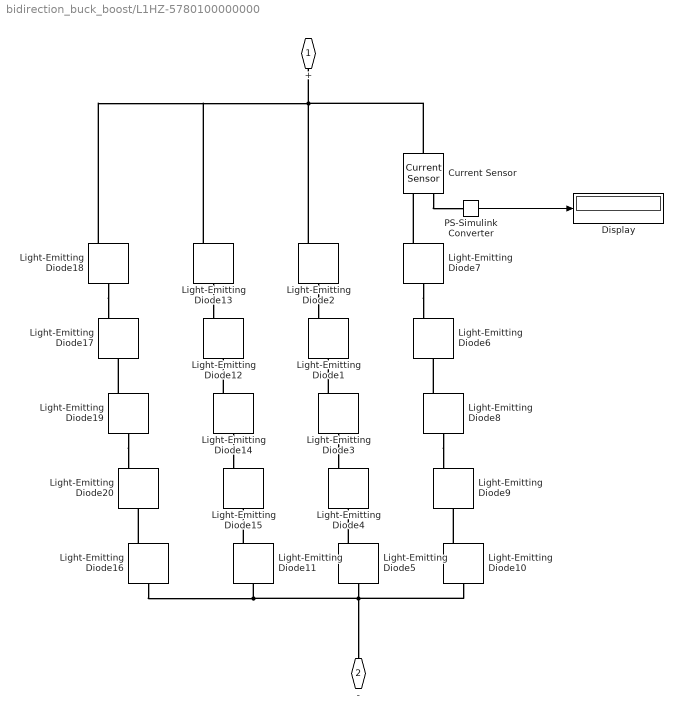
== system bidirection_buck_boost/L1HZ-5780100000000 ==
  Current Sensor : fl_lib/Electrical/Electrical Sensors/Current Sensor
  Display : Display
      settings: Format=bank
  Light-Emitting Diode{1..20} (20 alike) : ee_lib/Sensors & Transducers/Light-Emitting Diode  Gain=0.005 W/A  prmExp=ee.enum.diode.led.useIsN  I12=[.0017, .003] A  V12=[.9, 1.05] V  IS=3.3766e-22 A  ec=2.1758  RS=0.2718 Ohm  Tmeas=25 degC  C_param=ee.enum.diode.capParam.fixed  CJ=82.2 pF  CJ0=20 pF  Vvec=[.1, 10, 100] V  Cvec=[15, 10, 2] pF  VJ=1 V  Mgrad=0.5  FC=0.5  T_param=ee.enum.diode.temperatureParam.off  Tdevice=25 degC  IS_T2=1.8e-4 A  I1_T2=0.0034 A  V1_T2=1.05 V  Tmeas2=125 degC  EG_param=ee.enum.diode.egapParam.material_si  EG=1.11 eV  XTI_param=ee.enum.diode.xtiParam.pn  XTI=3  i_specify=off  i_priority=None  i=0 A  i_nominal_specify=off  i_nominal_value=1  i_nominal_unit=A  v_specify=off  v_priority=None  v=0 V  v_nominal_specify=off  v_nominal_value=1  v_nominal_unit=V  v_capacitor_specify=off  v_capacitor_priority=None  v_capacitor=0 V  v_capacitor_nominal_specify=off  v_capacitor_nominal_value=1  v_capacitor_nominal_unit=V  Qj_specify=off  Qj_priority=High  Qj=0 C  Qj_nominal_specify=off  Qj_nominal_value=1  Qj_nominal_unit=C  thermal_network_parameterization=ee.enum.thermalNetworkTopology.junctionCase  Rth=[0, 10] K/W  Rth_Cauer=[1, 3, 10] K/W  Rth_Foster=[.08, .14, .22, .16] K/W  thermal_mass_parameterization=ee.enum.thermalNetwork.timeconstant  thermal_mass=[0, 1] J/K  thermal_mass_Cauer=[1.5, 2, 3] J/K  thermal_mass_Foster=[.001, .005, .05, .5] J/K  thermal_time_constant=[0, 10] s  thermal_time_constant_Cauer=[1, 3, 10] s  thermal_time_constant_Foster=[7e-05, .0007, .01, .08] s  thermal_mass_initial_temperatures=[25, 25] degC  thermal_mass_initial_temperatures_Cauer=[25, 25, 25] degC  steadyState_Foster=simscape.enum.onoff.on  Tvec_initial_Foster=[25, 25, 25, 25] degC
      settings: InternalSimscapePortConfiguration="{\"Bottom\":[],\"Left\":[{\"id\":\"W\",\"label\":\"W\",\"type\":\"output\"},{\"id\":\"p\",\"label\":\"\",\"type\":\"foundation.electrical.electrical\"}],\"Right\":[{\"id\":\"n\",\"label\":\"\",\"type\":\"foundation.electrical.electrical\"}],\"Top\":[]}"
  PS-Simulink Converter : nesl_utility/PS-Simulink Converter  PhysicalDomain=network_engine_domain  SubClassName=ps_output  LeftPortType=input  RightPortType=output  PseudoPeriodic=off  Frequencies=[]  VectorFormat=inherit  Unit=inherit  AffineConversion=off
  + : PMIOPort  Side=Left
  - : PMIOPort  Port=2  Side=Right
  wires:
  PS-Simulink Converter/1 -> Display/1
  connections:
  Light-Emitting Diode5/RConn1 -- Light-Emitting Diode10/RConn1 -- Light-Emitting Diode16/RConn1 -- Light-Emitting Diode11/RConn1 -- -/RConn1
  Light-Emitting Diode7/LConn2 -- Current Sensor/RConn2
  Light-Emitting Diode5/LConn2 -- Light-Emitting Diode4/RConn1
  Light-Emitting Diode3/RConn1 -- Light-Emitting Diode4/LConn2
  Light-Emitting Diode3/LConn2 -- Light-Emitting Diode1/RConn1
  Light-Emitting Diode2/RConn1 -- Light-Emitting Diode1/LConn2
  Light-Emitting Diode7/RConn1 -- Light-Emitting Diode6/LConn2
  Light-Emitting Diode8/LConn2 -- Light-Emitting Diode6/RConn1
  Light-Emitting Diode8/RConn1 -- Light-Emitting Diode9/LConn2
  Light-Emitting Diode10/LConn2 -- Light-Emitting Diode9/RConn1
  Light-Emitting Diode11/LConn2 -- Light-Emitting Diode15/RConn1
  Light-Emitting Diode14/RConn1 -- Light-Emitting Diode15/LConn2
  Light-Emitting Diode14/LConn2 -- Light-Emitting Diode12/RConn1
  Light-Emitting Diode13/RConn1 -- Light-Emitting Diode12/LConn2
  Current Sensor/LConn1 -- Light-Emitting Diode18/LConn2 -- Light-Emitting Diode13/LConn2 -- Light-Emitting Diode2/LConn2 -- +/RConn1
  Current Sensor/RConn1 -- PS-Simulink Converter/LConn1
  Light-Emitting Diode18/RConn1 -- Light-Emitting Diode17/LConn2
  Light-Emitting Diode16/LConn2 -- Light-Emitting Diode20/RConn1
  Light-Emitting Diode19/RConn1 -- Light-Emitting Diode20/LConn2
  Light-Emitting Diode19/LConn2 -- Light-Emitting Diode17/RConn1

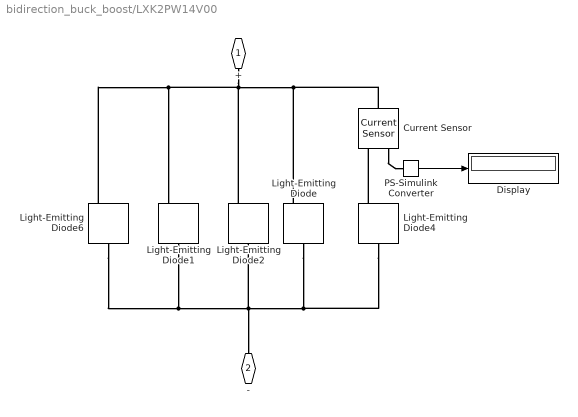
== system bidirection_buck_boost/LXK2PW14V00 ==
  Current Sensor : fl_lib/Electrical/Electrical Sensors/Current Sensor
  Display : Display
      settings: Format=bank
  Light-Emitting Diode{,1..2,4,6} (5 alike) : ee_lib/Sensors & Transducers/Light-Emitting Diode  Gain=0.005 W/A  prmExp=ee.enum.diode.led.useIsN  I12=[0.45833, 2.1666] A  V12=[2.8, 3.2] V  IS=3.5e-17 A  ec=3.12  RS=0.725 Ohm  Tmeas=25 degC  C_param=ee.enum.diode.capParam.fixed  CJ=1.2 nF  CJ0=x pF  Vvec=[.1, 10, 100] V  Cvec=[15, 10, 2] pF  VJ=1 V  Mgrad=0.5  FC=0.5  T_param=ee.enum.diode.temperatureParam.off  Tdevice=25 degC  IS_T2=1.8e-4 A  I1_T2=0.0034 A  V1_T2=1.05 V  Tmeas2=125 degC  EG_param=ee.enum.diode.egapParam.material_si  EG=1.11 eV  XTI_param=ee.enum.diode.xtiParam.pn  XTI=3  i_specify=off  i_priority=None  i=0 A  i_nominal_specify=off  i_nominal_value=1  i_nominal_unit=A  v_specify=off  v_priority=None  v=0 V  v_nominal_specify=off  v_nominal_value=1  v_nominal_unit=V  v_capacitor_specify=off  v_capacitor_priority=None  v_capacitor=0 V  v_capacitor_nominal_specify=off  v_capacitor_nominal_value=1  v_capacitor_nominal_unit=V  Qj_specify=off  Qj_priority=High  Qj=0 C  Qj_nominal_specify=off  Qj_nominal_value=1  Qj_nominal_unit=C  thermal_network_parameterization=ee.enum.thermalNetworkTopology.junctionCase  Rth=[0, 10] K/W  Rth_Cauer=[1, 3, 10] K/W  Rth_Foster=[.08, .14, .22, .16] K/W  thermal_mass_parameterization=ee.enum.thermalNetwork.timeconstant  thermal_mass=[0, 1] J/K  thermal_mass_Cauer=[1.5, 2, 3] J/K  thermal_mass_Foster=[.001, .005, .05, .5] J/K  thermal_time_constant=[0, 10] s  thermal_time_constant_Cauer=[1, 3, 10] s  thermal_time_constant_Foster=[7e-05, .0007, .01, .08] s  thermal_mass_initial_temperatures=[25, 25] degC  thermal_mass_initial_temperatures_Cauer=[25, 25, 25] degC  steadyState_Foster=simscape.enum.onoff.on  Tvec_initial_Foster=[25, 25, 25, 25] degC
      settings: InternalSimscapePortConfiguration="{\"Bottom\":[],\"Left\":[{\"id\":\"W\",\"label\":\"W\",\"type\":\"output\"},{\"id\":\"p\",\"label\":\"\",\"type\":\"foundation.electrical.electrical\"}],\"Right\":[{\"id\":\"n\",\"label\":\"\",\"type\":\"foundation.electrical.electrical\"}],\"Top\":[]}"
  PS-Simulink Converter : nesl_utility/PS-Simulink Converter  PhysicalDomain=network_engine_domain  SubClassName=ps_output  LeftPortType=input  RightPortType=output  PseudoPeriodic=off  Frequencies=[]  VectorFormat=inherit  Unit=inherit  AffineConversion=off
  + : PMIOPort  Side=Left
  - : PMIOPort  Port=2  Side=Right
  wires:
  PS-Simulink Converter/1 -> Display/1
  connections:
  Light-Emitting Diode1/RConn1 -- Light-Emitting Diode6/RConn1 -- Light-Emitting Diode2/RConn1 -- -/RConn1 -- Light-Emitting Diode/RConn1 -- Light-Emitting Diode4/RConn1
  Light-Emitting Diode2/LConn2 -- Light-Emitting Diode1/LConn2 -- Light-Emitting Diode6/LConn2 -- Current Sensor/LConn1 -- Light-Emitting Diode/LConn2 -- +/RConn1
  Light-Emitting Diode4/LConn2 -- Current Sensor/RConn2
  Current Sensor/RConn1 -- PS-Simulink Converter/LConn1

== matlab function bidirection_buck_boost/MATLAB Function1 ==
  data: Vs input; Is input; D output; S1_duty output; S1_NOT output; S2_duty output; S2_NOT output; Vout input; Iout input; Vout_ref input; Il input; S3_duty output; S3_NOT output; Ts input; discharge input; S4_duty output; S4_NOT output
function [D, S1_duty, S1_NOT, S2_duty, S2_NOT, S3_duty, S3_NOT, S4_duty, S4_NOT] = biDirBuckBoostController(Vs, Is, Vout, Iout, Vout_ref, Il, Ts, discharge)
% Bidirectional 4-switch DC-DC controller (MPPT + voltage limiting + buck-boost + current control + safe NOT outputs)
% PID/PI variables are defined globally for clarity
% Charging-specific variables are grouped under "CHARGING VARIABLES" section
% Discharge-specific variables are grouped under "DISCHARGE VARIABLES" section

%#codegen

%% ===================== GLOBAL / CHARGING VARIABLES =====================
% Safety / clamping
D_MAX = 0.92;
D_MIN = 0.1;
V_HYST_CHRG = 4.5; % hysteresis band (V)

% Voltage PI persistent
persistent v_int
if isempty(v_int), v_int = 0; end

% PID gains for voltage limiting (charging)
Kp_v_charging = 0.3;
Ki_v_charging = 35;

%% ===================== DISCHARGE VARIABLES =====================
persistent v_int_dis
if isempty(v_int_dis), v_int_dis = 0; end
persistent i_int_dis R_est_prev
if isempty(i_int_dis), i_int_dis = 0; end
if isempty(R_est_prev), R_est_prev = 3; end

%% ===================== INITIALIZE OUTPUTS =====================
D = 0.0;
S1_duty = 0.0; S1_NOT  = 1.0;
S2_duty = 0.0; S2_NOT  = 1.0;
S3_duty = 0.0; S3_NOT  = 1.0;
S4_duty = 0.0; S4_NOT  = 1.0;

%% ===================== CHARGE MODE CONTROL =====================
if discharge == 0
    if Vs > Vout - V_HYST_CHRG && Vs < Vout + V_HYST_CHRG
        % Buck-boost region: DC bus ≈ battery

        % --- MPPT duty ---
        D = mppt_p_and_o(Vs, Is);

        % --- Voltage limiting (PI) ---
        v_err = Vout_ref - Vout;
        if v_err < -V_HYST_CHRG
            v_int = v_int + Ki_v_charging * v_err * Ts;
        end
        D_voltage = D + Kp_v_charging * v_err + v_int;
        if D_voltage > D_MAX
            D = D_MAX; v_int = v_int - Ki_v_charging * v_err * Ts;
        elseif D_voltage < D_MIN
            D = D_MIN; v_int = v_int - Ki_v_charging * v_err * Ts;
        else
            D = D_voltage;
        end

        % --- Buck-boost switch mapping ---
        S1_duty = D;      S1_NOT  = 1.0;
        S2_duty = 0.0;    S2_NOT  = D;
        S3_duty = 0.0;    S3_NOT  = D;
        S4_duty = D;      S4_NOT  = 1.0;
        return;

    elseif Vs > Vout + V_HYST_CHRG
        % Buck region: DC bus > battery
        D = mppt_p_and_o(Vs, Is);
        v_err = Vout_ref - Vout;
        if v_err < -V_HYST_CHRG
            v_int = v_int + Ki_v_charging * v_err * Ts;
        end
        D_voltage = D + Kp_v_charging * v_err + v_int;
        if D_voltage > D_MAX
            D = D_MAX; v_int = v_int - Ki_v_charging * v_err * Ts;
        elseif D_voltage < D_MIN
            D = D_MIN; v_int = v_int - Ki_v_charging * v_err * Ts;
        else
            D = D_voltage;
        end
        % --- Buck switch mapping ---
        S1_duty = D;      S1_NOT  = 1.0;
        S2_duty = 0.0;    S2_NOT  = D;
        S3_duty = 1.0;    S3_NOT  = 1.0;
        S4_duty = 0.0;    S4_NOT  = 1.0;
        return;
    end
end

%% ===================== DISCHARGE MODE CONTROL (VOLTAGE + CURRENT HYSTERESIS) =====================
if discharge == 1
    % ----- Reference & limits -----
    % For led - LXK2PW14V00
    % Vref_led      = 4.2;       % desired LED voltage (V)
    % V_HYST_DISCH  = 0.35;        % voltage hysteresis band (V)
    % I_target_nom  = 7.2;        % nominal LED current (A)
    % I_abs_max     = 8.0;        % max allowed current (A)
    % I_HYST_DISCH  = 0.03;       % current hysteresis (A)
    
    % For led - L1HZ-5780100000000
    Vref_led      = 14.4;       % desired LED voltage (V)
    V_HYST_DISCH  = 0.50;        % voltage hysteresis band (V)
    I_target_nom  = 1.0;        % nominal LED current (A)
    I_abs_max     = 1.4;        % max allowed current (A)
    I_HYST_DISCH  = 0.01;       % current hysteresis (A)


    % ----- Gains -----
    Kp_v = 0.12;   Ki_v = 40;   % outer voltage PI
    Kp_i = 0.45;   Ki_i = 270;  % inner current PI
    FF_mix = 0.6;               % feedforward weighting

    % ----- Measured variables -----
    I_load = -Is;               % A (positive during discharge)
    V_load = Vs;                % V (load/LED voltage)
    V_batt = Vout;              % V (battery)

    % ================= OUTER VOLTAGE LOOP (hysteretic) =================
    v_err = Vref_led - V_load;


    % Apply hysteresis: only integrate when outside deadband
    if abs(v_err) > V_HYST_DISCH
        v_int_dis = v_int_dis + Ki_v * v_err * Ts;
    end
    % anti-windup clamp
    v_int_dis = min(max(v_int_dis, -1.0), 1.0);

    % voltage controller output -> current reference
    I_target = Kp_v * v_err + v_int_dis + I_target_nom;
    % limit to physical range
    I_target = min(max(I_target, 0.0), I_abs_max);

    % ================= INNER CURRENT LOOP =================
    % Feed-forward estimate of duty from R estimate
    epsI = 1e-4;
    R_inst = V_load / max(I_load, epsI);
    alphaR = 0.08;
    R_est = (1 - alphaR) * R_est_prev + alphaR * R_inst;
    R_est_prev = R_est;

    V_load_ff = I_target * R_est;
    if V_load_ff <= V_batt
        D_ff = V_load_ff / max(V_batt, 1e-6);     % buck
    else
        D_ff = 1 - (V_batt / max(V_load_ff, 1e-6)); % boost
    end
    D_ff = min(max(D_ff, D_MIN), D_MAX);

    % Current PI

    if isempty(i_int_dis), i_int_dis = 0; end
    i_err = I_target - I_load;

    if abs(i_err) > I_HYST_DISCH
        i_int_dis = i_int_dis + Ki_i * i_err * Ts;
    end
    % clamp integrator
    i_int_dis = min(max(i_int_dis, -0.6), 0.6);

    D_corr = Kp_i * i_err + i_int_dis;

    % Combine FF + correction
    D_unsat = FF_mix * D_ff + (1 - FF_mix) * (D_ff + D_corr);

    % Saturation + anti-windup
    if D_unsat > D_MAX
        D = D_MAX;
        i_int_dis = i_int_dis - Ki_i * i_err * Ts;
    elseif D_unsat < D_MIN
        D = D_MIN;
        i_int_dis = i_int_dis - Ki_i * i_err * Ts;
    else
        D = D_unsat;
    end

    % ================= SAFETY LIMITS =================
    if I_load > (I_abs_max + I_HYST_DISCH)
        D = max(D_MIN, D * 0.5);
        i_int_dis = 0;
    end

    % ================= SWITCH MAPPING =================
    if Vs > Vout + V_HYST_CHRG
        % Boost region
        S1_duty = 0;  S1_NOT = D;
        S2_duty = D;  S2_NOT = 1;
        S3_duty = 1;  S3_NOT = 1;
        S4_duty = 0;  S4_NOT = 1;
    elseif Vs < Vout - V_HYST_CHRG
        % Buck region
        S1_duty = 1;  S1_NOT = 1;
        S2_duty = 0;  S2_NOT = 1;
        S3_duty = D;  S3_NOT = 1;
        S4_duty = 0;  S4_NOT = D;
    else
        % Buck-boost transition
        S1_duty = 0;  S1_NOT = D;
        S2_duty = D;  S2_NOT = 1;
        S3_duty = D;  S3_NOT = 1;
        S4_duty = 0;  S4_NOT = D;
    end

    return;
end




%% ===================== DEFAULT / SAFE OUTPUTS =====================
D = 0.0;
S1_duty = 0.0; S1_NOT  = 1.0;
S2_duty = 0.0; S2_NOT  = 1.0;
S3_duty = 0.0; S3_NOT  = 1.0;
S4_duty = 0.0; S4_NOT  = 1.0;
return;

%% --------------------------------------------------------------------
%% Nested helper: Perturb & Observe MPPT (codegen friendly)
%% --------------------------------------------------------------------
function Dout = mppt_p_and_o(V, I)
    %#codegen
    persistent V_old P_old D_old initialized;
    if isempty(initialized)
        V_old = V; P_old = V*I; D_old = 0.5; initialized = true; Dout = D_old; return;
    end
    DEL_D = 0.002;
    D_MAX_local = D_MAX; D_MIN_local = D_MIN;
    P_new = V*I; dV = V - V_old; dP = P_new - P_old;
    if dP > 0
        if dV > 0, D = D_old - DEL_D; else, D = D_old + DEL_D; end
    elseif dP < 0
        if dV > 0, D = D_old + DEL_D; else, D = D_old - DEL_D; end
    else
        D = D_old;
    end
    if D > D_MAX_local, D = D_MAX_local; elseif D < D_MIN_local, D = D_MIN_local; end
    D_old = D; V_old = V; P_old = P_new;
    Dout = D;
end

end
